simulink model "SixDOFSim"  (R2026b)
settings: Solver=VariableStepAuto  StopTime=400
values from neighbouring files (symbols this model uses):
  A = [A_1 zeros(n/2,n/2);zeros(n/2,n/2) A_2]    [defineABC.m]    (also in implicit_linmod.m = -inv(E)*A_prime; nonlinear_6DOF.m = q_d*S*CA; normieren.m = Tx\A*Tx)
  B = [B_1, zeros(n/2,m/2);zeros(n/2,m/2), B_2]    [defineABC.m]    (also in implicit_linmod.m = -inv(E)*B_prime; normieren.m = Tx\B*Tu)
  C = zeros(m,n)    [defineABC.m]    (also in normieren.m = (Ty\C*Tx))
  eta_max = 10*pi/180    (= 0.174532925199)    [SixDOFModel.m]
  eta_min = - 25*pi/180    (= -0.436332312999)    [SixDOFModel.m]
  F = -inv(C*(Ak\B))    [SixDOFModel.m]    (also in coupling_controller.m = Kopt{end}; implicit_linmod.m = feval(fun, dX_ap, X_ap, U_minus))
  I_inv = inv(I)    [initializeParameters.m]
  K = lqr(sys_ol,Q,R)    [SixDOFModel.m]
  latlon_init = [0;0]    [SixDOFModel.m]
  m = size(B_1,2) + size(B_2,2)    [defineABC.m]    (also in implicit_linmod.m = length(U_ap); initializeParameters.m = 120000)
  n = size(A_1,1) +size(A_2,2)    [defineABC.m]    (also in implicit_linmod.m = length(X_ap); normieren.m = size(A,2))
  Omega_init_1 = [0;0;0]    [SixDOFModel.m]
  Omega_init_2 = [0;0;0]    [SixDOFModel.m]
  P_e_init_1 = [0;0;-h_init_1]    [SixDOFModel.m]
  P_e_init_2 = [0;0;-h_init_2]    [SixDOFModel.m]
  Phi_init_1 = [0;0;0]    [SixDOFModel.m]
  Phi_init_2 = [0;0;0]    [SixDOFModel.m]
  sigmaf_max = 10*pi/180    (= 0.174532925199)    [SixDOFModel.m]
  sigmaf_min = 0.5*pi/180    (= 0.00872664625997)    [SixDOFModel.m]
  U_ap = [U_ap_1;U_ap_2]    [SixDOFModel.m]    (also in trimValues.m = Z_ap(11:14))
  U_test = [-0.12;1;0;0;-0.1;1;0;0]    [SixDOFModel.m]
  V_init_1 = [200;0;0]    [SixDOFModel.m]
  V_init_2 = [220;0;0]    [SixDOFModel.m]
  W_ap = [X_ap_1(1); X_ap_2(1); 0; 0; X_ap_1(10); X_ap_2(10); 0; 0]    [SixDOFModel.m]
  X_ap = [X_ap_1;X_ap_2]    [SixDOFModel.m]    (also in trimValues.m = Z_ap(1:10))
  X_init = [X_init_1;X_init_2]    [SixDOFModel.m]
  xi_max = 25*pi/180    (= 0.436332312999)    [SixDOFModel.m]
  xi_min = - xi_max    (= -0.436332312999)    [SixDOFModel.m]
  zita_max = 30*pi/180    (= 0.523598775598)    [SixDOFModel.m]
  zita_min = - zita_max    (= -0.523598775598)    [SixDOFModel.m]
undefined symbols (not defined in the file or in its folder): Earth, globalParameters, nonlinear_6DOF, WGS84
libraries: aerolibfltsims x38, aerolibtransform2 x6, aerolibwind2 x2, simulink x2, aerolibatmos2 x2
(part 3 of 3)

== matlab function SixDOFSim/6 DOF Model Boeing 757 200/Motion model Plain2 /Dynamics/Transformation of gravity in (Körperfestes System) ==
  data: Phi input; gravityAcceleration output; g parameter
function gravityAcceleration = Tfg(Phi,g)
G_geod = [0;0;g]; %Graviation vector in geodetic ref. Frame
Tfg = coordTransfMatrix(Phi(1),1)*coordTransfMatrix(Phi(2),2)*coordTransfMatrix(Phi(3),3); % Transformation Matrix goedetic --> body reference Frame
gravityAcceleration = Tfg*G_geod;

== matlab function SixDOFSim/6 DOF Model Boeing 757 200/Geometrical Coefficients Plane 1/Geometry Translational Coefficients ==
  data: vA input; alpha input; CA output; beta input; Omega input; globalParameters parameter; CW output; CQ output; eta input; zita input
function [CA,CW,CQ] = forceGeometryCoefficients(vA,alpha,beta,Omega,globalParameters,eta,zita)
%eta = Höheruderwinkel (elevator) [rad]
%zita = Seitenruderwinkel (ruder) [rad]
%Global Parameters
lt = globalParameters.lt;
S = globalParameters.S;
St = globalParameters.St;
% Rotration rates [rad/s]
q = Omega(2); %Nickrate (Pitch Rate)
%Constants Coefficients
grad_alpha = 5.5;
alpha_L0 = -11.5*pi/180;
gradient_alpha_epsolon = 0.25;
gradient_CQ_Cbeta = -1.6;
gradientCQ_Czita = 0.24;
CW0 = 0.13;
kappa = 0.07;
a3 = -768.5;
a2 = 609.2;
a1 = -155.2;
a0 = 15.212;
%Forces Coefficients
if alpha <=14.5*pi/180
     
     CA_F = grad_alpha*(alpha -alpha_L0);
else
     CA_F = a3*alpha^.3+a2*alpha^.2+a1*alpha +a0;% Lift Coefficient without the Control Aereas
end
epsolon = gradient_alpha_epsolon*(alpha - alpha_L0); %Downwash [rad]
alpha_t = alpha - epsolon + eta +1.3*q*lt/vA; %Angle of Attack of the Tail [rad]
CA_H = 3.1*(St/S)*alpha_t; %Lift Coefficient of the Control Aereas (Elevator-Tail)
CA = CA_F + CA_H; %Total Lift Coefficient
CW = CW0 + kappa*(5.5*alpha + 0.654)^2; %Drag Coefficient
CQ = gradient_CQ_Cbeta*beta + gradientCQ_Czita*zita;

== matlab function SixDOFSim/6 DOF Model Boeing 757 200/Motion model Plain2 /Kinematics/Rotation Rate of the g-System ==
  data: Omega input; dPhi output; Phi input
function dPhi = J(Omega,Phi)
%Rotation rate of the g-system depending on the euler angles
%Phi: euler Angles
%Omega_ diff = Omega-Omega_g
%dPhi: Rotaion Speed considering the rotation rate of the geodathic system
phi = Phi(1);
theta = Phi(2);
J = 1/cos(theta)*[cos(theta) sin(phi)*sin(theta) cos(phi)*sin(theta) ;0 cos(phi)*cos(theta) -sin(phi)*cos(theta);0 sin(phi) cos(phi)]; %Rotation rate matrix
dPhi = J*Omega;

== matlab function SixDOFSim/6 DOF Model Boeing 757 200/Motion model Plain2 /Kinematics/Velocity Transformation to Erdfestkoordinaten ==
  data: Phi input; V input; velocityDEN output
function velocityDEN = Tgf(Phi,V)
%Converts the velocity from Körper to Erdfest Koordinaten
%Phi: Vector w. Euler Angles
% P_erdfest: Position Vector 
phi = Phi(1);
theta = Phi(2);
psi = Phi(3);
Tfg =  coordTransfMatrix(phi,1)*coordTransfMatrix(theta,2)*coordTransfMatrix(psi,3); % Transformation Matrix goedetic --> body reference Frame
Tgf = Tfg';%Transformation to North East Down
velocityDEN = Tgf*V;

== matlab function SixDOFSim/6 DOF Model Boeing 757 200/Motion model Plain2 /MATLAB Function ==
  data: P_e input; h output
function h = getHeight(P_e)
h = - P_e(3);

== matlab function SixDOFSim/6 DOF Model Boeing 757 200/Motion model Plain2 /Track and Aerodynamical Speed ==
  data: Phi input; V input; vk output; vA output; alpha output; beta output; Vw_geod input; gamma output; chsi output
function [vk,vA,alpha,beta,gamma,chsi] = getTrackAndAero(Phi,V,Vw_geod)
%Get The Track Speed, the Approach Speed, the inclinational angle ,
%the Azimuth angle, the angle of attack and the Sliding angle from the
%Speed from the Translational Velocity. 
Tfg = coordTransfMatrix(Phi(1),1)*coordTransfMatrix(Phi(2),2)*coordTransfMatrix(Phi(3),3); % Transformation Matrix goedetic --> body reference Frame
Tgf = Tfg';
Vk = Tgf*V; %Track Velocity
vk = sqrt(Vk(1)^2+Vk(2)^2+Vk(3)^2); %Track Speed [m/s]
gamma = -asin(Vk(3)/vk); %Inclination Angle [rad]
chsi = atan2(Vk(2),Vk(1));
Vw = Tfg*Vw_geod;
VA = V - Vw; %Approach Speed
vA = sqrt(VA(1)^2+VA(2)^2+VA(3)^2); %Approach Speed [m/s]
alpha = atan(VA(3)/VA(1)); % Angle of attck [m/s]
beta = asin(VA(2)/vA);
% dvA = (VA(1)*dV(1) + VA(2)*dV(2) +VA(3)*dV(3))/(vA); %Derivative of the Approach Speed
% dalpha = (dV(3)*VA(1)-dV(1)*VA(3))/(VA(1)^2+VA(1)*VA(3)); %Derivative of Angle of Attack
% dbeta = (dV(2)*vA -dvA*VA(2))/(vA*sqrt(vA^2-VA(2)^2)); %Derivative of Sideslip Angle

== matlab function SixDOFSim/6 DOF Model Boeing 757 200/MATLAB Function1 ==
  data: Phi input; DCM output
function DCM = getTfg(Phi)

DCM = coordTransfMatrix(Phi(1),1)*coordTransfMatrix(Phi(2),2)*coordTransfMatrix(Phi(3),3); % Transformation Matrix goedetic --> body reference Frame

== matlab function SixDOFSim/6 DOF Model Boeing 757 200/Motion model Plain1/Dynamics/Dynamics Forces Feedback ==
  data: Omega input; V input; acceleration output; globalParameters parameter
function acceleration = accelerationFeedback(Omega,V,globalParameters)
Omega_e_tilde = globalParameters.Omega_e_tilde;
Omega_tilde = vecToMat(Omega);
acceleration = (Omega_tilde + Omega_e_tilde)*V;

== matlab function SixDOFSim/6 DOF Model Boeing 757 200/Motion model Plain1/Dynamics/Dynamics Torque Feedback ==
  data: Omega input; torqueFeedback output; globalParameters parameter
function torqueFeedback = getTorqueFeedback(Omega,globalParameters)
I = globalParameters.I;
Omega_tilde = vecToMat(Omega);
help = Omega_tilde*I;
torqueFeedback = help*Omega;

== matlab function SixDOFSim/6 DOF Model Boeing 757 200/Motion model Plain1/Dynamics/Transformation of gravity in (Körperfestes System) ==
  data: Phi input; gravityAcceleration output; g parameter
function gravityAcceleration = Tfg(Phi,g)
G_geod = [0;0;g]; %Graviation vector in geodetic ref. Frame
Tfg = coordTransfMatrix(Phi(1),1)*coordTransfMatrix(Phi(2),2)*coordTransfMatrix(Phi(3),3); % Transformation Matrix goedetic --> body reference Frame
gravityAcceleration = Tfg*G_geod;

== matlab function SixDOFSim/6 DOF Model Boeing 757 200/Motion model Plain1/Kinematics/Rotation Rate of the g-System ==
  data: Omega input; dPhi output; Phi input
function dPhi = J(Omega,Phi)
%Rotation rate of the g-system depending on the euler angles
%Phi: euler Angles
%Omega_ diff = Omega-Omega_g
%dPhi: Rotaion Speed considering the rotation rate of the geodathic system
phi = Phi(1);
theta = Phi(2);
J = 1/cos(theta)*[cos(theta) sin(phi)*sin(theta) cos(phi)*sin(theta) ;0 cos(phi)*cos(theta) -sin(phi)*cos(theta);0 sin(phi) cos(phi)]; %Rotation rate matrix
dPhi = J*Omega;

== matlab function SixDOFSim/6 DOF Model Boeing 757 200/Motion model Plain1/Kinematics/Velocity Transformation to Erdfestkoordinaten ==
  data: Phi input; V input; velocityDEN output
function velocityDEN = Tgf(Phi,V)
%Converts the velocity from Körper to Erdfest Koordinaten
%Phi: Vector w. Euler Angles
% P_erdfest: Position Vector 
phi = Phi(1);
theta = Phi(2);
psi = Phi(3);
Tfg =  coordTransfMatrix(phi,1)*coordTransfMatrix(theta,2)*coordTransfMatrix(psi,3); % Transformation Matrix goedetic --> body reference Frame
Tgf = Tfg';%Transformation to North East Down
velocityDEN = Tgf*V;

== matlab function SixDOFSim/6 DOF Model Boeing 757 200/Motion model Plain1/MATLAB Function ==
  data: P_e input; h output
function h = getHeight(P_e)
h = - P_e(3);

== matlab function SixDOFSim/6 DOF Model Boeing 757 200/Motion model Plain1/Track and Aerodynamical Speed ==
  data: Phi input; V input; vk output; vA output; alpha output; beta output; Vw_geod input; gamma output; chsi output
function [vk,vA,alpha,beta,gamma,chsi] = getTrackAndAero(Phi,V,Vw_geod)
%Get The Track Speed, the Approach Speed, the inclinational angle ,
%the Azimuth angle, the angle of attack and the Sliding angle from the
%Speed from the Translational Velocity. 
Tfg = coordTransfMatrix(Phi(1),1)*coordTransfMatrix(Phi(2),2)*coordTransfMatrix(Phi(3),3); % Transformation Matrix goedetic --> body reference Frame
Tgf = Tfg';
Vk = Tgf*V; %Track Velocity
vk = sqrt(Vk(1)^2+Vk(2)^2+Vk(3)^2); %Track Speed [m/s]
gamma = -asin(Vk(3)/vk); %Inclination Angle [rad]
chsi = atan2(Vk(2),Vk(1));
Vw = Tfg*Vw_geod;
VA = V - Vw; %Approach Speed
vA = sqrt(VA(1)^2+VA(2)^2+VA(3)^2); %Approach Speed [m/s]
alpha = atan(VA(3)/VA(1)); % Angle of attck [m/s]
beta = asin(VA(2)/vA);
% dvA = (VA(1)*dV(1) + VA(2)*dV(2) +VA(3)*dV(3))/(vA); %Derivative of the Approach Speed
% dalpha = (dV(3)*VA(1)-dV(1)*VA(3))/(VA(1)^2+VA(1)*VA(3)); %Derivative of Angle of Attack
% dbeta = (dV(2)*vA -dvA*VA(2))/(vA*sqrt(vA^2-VA(2)^2)); %Derivative of Sideslip Angle

== matlab function SixDOFSim/6 DOF Non Linear Model Equations/Visualisation Non Linear Model 2/Body to Earth Reference Frame  ==
  data: V input; Phi input; V_e output
function V_e = getEarthPosition(V,Phi)

Tfg = coordTransfMatrix(Phi(1),1)*coordTransfMatrix(Phi(2),2)*coordTransfMatrix(Phi(3),3); % Transformation Matrix goedetic --> body reference Frame
Tgf = Tfg';
V_e = Tgf*V;
V_e(3) =  V_e(3);

== matlab function SixDOFSim/6 DOF Non Linear Model Equations/Visualisation Non Linear Model 2/MATLAB Function ==
  data: V input; vA output; alpha output; beta output
function [vA,alpha,beta] = getAerodynamical(V)
u = V(1);
v = V(2);
w = V(3);
vA = sqrt(u^2+v^2+w^2);
alpha = atan2(w,u);
beta = asin(v/vA);

== matlab function SixDOFSim/6 DOF Linear/Visualisation Non Linear Model Plain 1/Body to Earth Reference Frame  ==
  data: V input; Phi input; V_e output
function V_e = getEarthPosition(V,Phi)

Tfg = coordTransfMatrix(Phi(1),1)*coordTransfMatrix(Phi(2),2)*coordTransfMatrix(Phi(3),3); % Transformation Matrix goedetic --> body reference Frame
Tgf = Tfg';
V_e = Tgf*V;
V_e(3) =  V_e(3);

== matlab function SixDOFSim/6 DOF Model Boeing 757 200/Geometrical Coefficients Plain2/Geometry Translational Coefficients ==
  data: vA input; alpha input; CA output; beta input; Omega input; globalParameters parameter; CW output; CQ output; eta input; zita input
function [CA,CW,CQ] = forceGeometryCoefficients(vA,alpha,beta,Omega,globalParameters,eta,zita)
%eta = Höheruderwinkel (elevator) [rad]
%zita = Seitenruderwinkel (ruder) [rad]
%Global Parameters
lt = globalParameters.lt;
S = globalParameters.S;
St = globalParameters.St;
% Rotration rates [rad/s]
q = Omega(2); %Nickrate (Pitch Rate)
%Constants Coefficients
grad_alpha = 5.5;
alpha_L0 = -11.5*pi/180;
gradient_alpha_epsolon = 0.25;
gradient_CQ_Cbeta = -1.6;
gradientCQ_Czita = 0.24;
CW0 = 0.13;
kappa = 0.07;
a3 = -768.5;
a2 = 609.2;
a1 = -155.2;
a0 = 15.212;
%Forces Coefficients
if alpha <=14.5*pi/180
     
     CA_F = grad_alpha*(alpha -alpha_L0);
else
     CA_F = a3*alpha^.3+a2*alpha^.2+a1*alpha +a0;% Lift Coefficient without the Control Aereas
end
epsolon = gradient_alpha_epsolon*(alpha - alpha_L0); %Downwash [rad]
alpha_t = alpha - epsolon + eta +1.3*q*lt/vA; %Angle of Attack of the Tail [rad]
CA_H = 3.1*(St/S)*alpha_t; %Lift Coefficient of the Control Aereas (Elevator-Tail)
CA = CA_F + CA_H; %Total Lift Coefficient
CW = CW0 + kappa*(5.5*alpha + 0.654)^2; %Drag Coefficient
CQ = gradient_CQ_Cbeta*beta + gradientCQ_Czita*zita;

== matlab function SixDOFSim/6 DOF Linear/Visualisation Non Linear Model Plain 1/MATLAB Function ==
  data: V input; vA output; alpha output; beta output
function [vA,alpha,beta] = getAerodynamical(V)
u = V(1);
v = V(2);
w = V(3);
vA = sqrt(u^2+v^2+w^2);
alpha = atan2(w,u);
beta = asin(v/vA);

== matlab function SixDOFSim/6 DOF Non Linear Model Equations1/Visualisation Non Linear Model 1/Body to Earth Reference Frame  ==
  data: V input; Phi input; V_e output
function V_e = getEarthPosition(V,Phi)

Tfg = coordTransfMatrix(Phi(1),1)*coordTransfMatrix(Phi(2),2)*coordTransfMatrix(Phi(3),3); % Transformation Matrix goedetic --> body reference Frame
Tgf = Tfg';
V_e = Tgf*V;
V_e(3) =  V_e(3);

== matlab function SixDOFSim/6 DOF Non Linear Model Equations1/Visualisation Non Linear Model 1/MATLAB Function ==
  data: V input; vA output; alpha output; beta output
function [vA,alpha,beta] = getAerodynamical(V)
u = V(1);
v = V(2);
w = V(3);
vA = sqrt(u^2+v^2+w^2);
alpha = atan2(w,u);
beta = asin(v/vA);

== matlab function SixDOFSim/6 DOF Non Linear Model Equations1/Visualisation Non Linear Model 2/Body to Earth Reference Frame  ==
  data: V input; Phi input; V_e output
function V_e = getEarthPosition(V,Phi)

Tfg = coordTransfMatrix(Phi(1),1)*coordTransfMatrix(Phi(2),2)*coordTransfMatrix(Phi(3),3); % Transformation Matrix goedetic --> body reference Frame
Tgf = Tfg';
V_e = Tgf*V;
V_e(3) =  V_e(3);

== matlab function SixDOFSim/6 DOF Non Linear Model Equations1/Visualisation Non Linear Model 2/MATLAB Function ==
  data: V input; vA output; alpha output; beta output
function [vA,alpha,beta] = getAerodynamical(V)
u = V(1);
v = V(2);
w = V(3);
vA = sqrt(u^2+v^2+w^2);
alpha = atan2(w,u);
beta = asin(v/vA);

== matlab function SixDOFSim/6 DOF Non Linear Model Equations/Visualisation Non Linear Model 1/Body to Earth Reference Frame  ==
  data: V input; Phi input; V_e output
function V_e = getEarthPosition(V,Phi)

Tfg = coordTransfMatrix(Phi(1),1)*coordTransfMatrix(Phi(2),2)*coordTransfMatrix(Phi(3),3); % Transformation Matrix goedetic --> body reference Frame
Tgf = Tfg';
V_e = Tgf*V;
V_e(3) =  V_e(3);

== matlab function SixDOFSim/6 DOF Non Linear Model Equations/Visualisation Non Linear Model 1/MATLAB Function ==
  data: V input; vA output; alpha output; beta output
function [vA,alpha,beta] = getAerodynamical(V)
u = V(1);
v = V(2);
w = V(3);
vA = sqrt(u^2+v^2+w^2);
alpha = atan2(w,u);
beta = asin(v/vA);

== matlab function SixDOFSim/6 DOF Model Boeing 757 200/Forces and Moments Plane 1/Aerodynamical Forces ==
  data: CA input; RA output size=3; CW input; CQ input; vA input; alpha input; beta input; rho input; globalParameters parameter
function RA = getAerodynForces(CA,CW,CQ,vA, alpha, beta, rho,globalParameters)

q_d = 0.5*vA^2*rho; %Dynamic Preassure
S = globalParameters.S ;


A = q_d*S*CA; %Lift Force [N]
W = q_d*S*CW; %Air Resistance [N]
Q = q_d*S*CQ; %Transverse Force [N]

Tfa = coordTransfMatrix(alpha,2)*coordTransfMatrix(-beta,3); %Transformation Matrix Aerodynamics -> Körperfest

RA_a =[-W;Q;-A];
RA = Tfa*RA_a;

== matlab function SixDOFSim/6 DOF Model Boeing 757 200/Forces and Moments Plane 1/Aerodynamical Torque ==
  data: RA input; CL input; QA output size=3; CM input; CN input; vA input; globalParameters parameter; rho input
function QA = getAerodynTorque(RA,CL,CM,CN, vA, globalParameters,rho)
% h = P_e(3); %Height [m]
% [~,~,~,rho] = atmosisa(h); %Air density 
%Aircraft Parameters
b = globalParameters.b;
%rho = globalParameters.rho;
c = globalParameters.c;
S = globalParameters.S;
P_centerGravity = globalParameters.P_centerGravity;
P_aerodynCenter = globalParameters.P_aerodynCenter;
q_d = 0.5*vA^2*rho; %Dynamic Preassure


QA_aerodynCenter = q_d*S*[0.5*b*CL;c*CM;0.5*b*CN];
QA = QA_aerodynCenter + vecToMat(P_centerGravity- P_aerodynCenter)*RA;

== matlab function SixDOFSim/6 DOF Model Boeing 757 200/MATLAB Function2 ==
  data: Phi input; DCM output
function DCM = getTfg(Phi)

DCM = coordTransfMatrix(Phi(1),1)*coordTransfMatrix(Phi(2),2)*coordTransfMatrix(Phi(3),3); % Transformation Matrix goedetic --> body reference Frame
